simulink model "PID_Motor_Control"  (R2025b)
settings: Solver=VariableStepAuto  StartTime=0.0  StopTime=10.0  RelTol=1e-3
model workspace (MAT data in the model file):
  Kd = Simulink.Parameter
  Kd.Value = 0
  Kd.Complexity = 'real'
  Kd.Dimensions = [1 1]
  Kd.DataType = 'auto'
  Ki = Simulink.Parameter
  Ki.Value = 0
  Ki.Complexity = 'real'
  Ki.Dimensions = [1 1]
  Ki.DataType = 'auto'
  Km = Simulink.Parameter
  Km.Value = 11661
  Km.Complexity = 'real'
  Km.Dimensions = [1 1]
  Km.DataType = 'auto'
  Kp = Simulink.Parameter
  Kp.Value = 0.08
  Kp.Complexity = 'real'
  Kp.Dimensions = [1 1]
  Kp.DataType = 'auto'
  Setpoint = Simulink.Parameter
  Setpoint.Value = 500
  Setpoint.Complexity = 'real'
  Setpoint.Dimensions = [1 1]
  Setpoint.DataType = 'auto'
  Tm = Simulink.Parameter
  Tm.Value = 0.017
  Tm.Complexity = 'real'
  Tm.Dimensions = [1 1]
  Tm.DataType = 'auto'
settings Model: Creator=grantdahl  LastModifiedBy=grantdahl

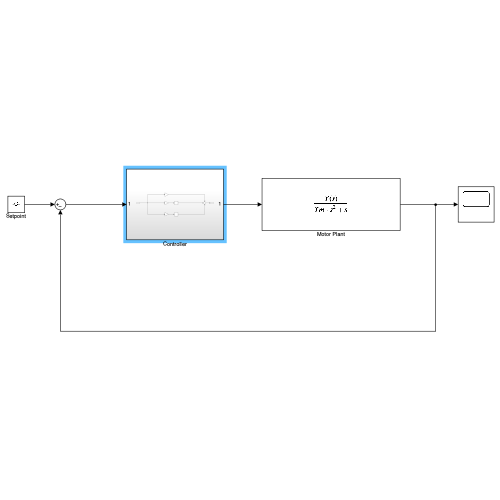
[thumbnail: Simulink's stored preview of the top-level diagram]
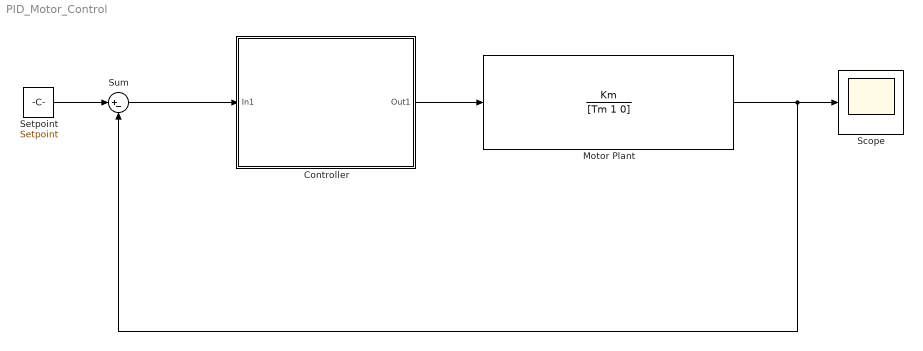
== system PID_Motor_Control ==
  Controller : Subsystem
  Motor Plant : TransferFcn  Numerator=Km  Denominator=[Tm 1 0]
  Scope : Scope
      settings: ActiveDisplayYMinimum=491.80861070390597  ActiveDisplayYMaximum=513.76743963911792
  Setpoint : Constant  Value=Setpoint
  Sum : Sum  Inputs=|+-
  wires:
  Controller/1(Out1) -> Motor Plant/1
  Motor Plant/1 -> Sum/2, Scope/1
  Sum/1 -> Controller/1(In1)
  Setpoint/1 -> Sum/1

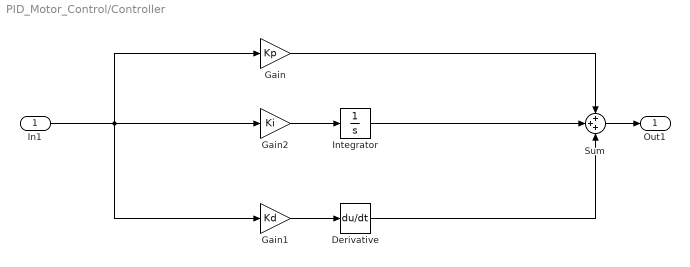
== system PID_Motor_Control/Controller ==
  In1 : Inport
  Derivative : Derivative
  Gain : Gain  Gain=Kp
  Gain1 : Gain  Gain=Kd
  Gain2 : Gain  Gain=Ki
  Integrator : Integrator
  Sum : Sum  Inputs=+++
  Out1 : Outport
  wires:
  Sum/1 -> Out1/1
  In1/1 -> Gain2/1, Gain1/1, Gain/1
  Integrator/1 -> Sum/2
  Gain/1 -> Sum/1
  Gain1/1 -> Derivative/1
  Gain2/1 -> Integrator/1
  Derivative/1 -> Sum/3
